simulink model "levitador_bola"  (R2023b)
settings: Solver=ode45  StartTime=0.0  StopTime=t_final  MaxStep=Ts/8  RelTol=1e-3
values from neighbouring files (symbols this model uses):
  folga = 45    [parametros_levitador.m]
  g = 9.81    [parametros_levitador.m]
  h_eq = [0     0.017 0.080 0.103 0.138 0.157 0.22 ]    [parametros_levitador.m]
  h_ini = 0.13    [parametros_levitador.m]
  K_v = 0.0063    [parametros_levitador.m]
  Kd = 250    [parametros_levitador.m]
  Ki = 5    [parametros_levitador.m]
  Kp = 130    [parametros_levitador.m]
  N_filtro = 25    [parametros_levitador.m]
  pwm_eq = [143.6 141.1 133.2 129.0 126.7 127.3 127.3]    [parametros_levitador.m]
  ruido_s = rd0    [analise_levitador.m]    (also in parametros_levitador.m = 6.25e-06)
  semente = 10*sem    [comparar_candidatos.m]    (also in parametros_levitador.m = 1)
  tau_v = 0.56    [parametros_levitador.m]
  Ts = 0.04    [parametros_levitador.m]
  turb_f = 0    [parametros_levitador.m]
  turb_sd = sd0    [analise_levitador.m]    (also in parametros_levitador.m = 4)
  u0 = 127    [parametros_levitador.m]
  u_max = 255    [parametros_levitador.m]
  u_min = 0    [parametros_levitador.m]
  v_ar_ini = K_v*pwm0    [parametros_levitador.m]
libraries: slpidlib x1
settings Model: Creator=autor  LastModifiedBy=autor

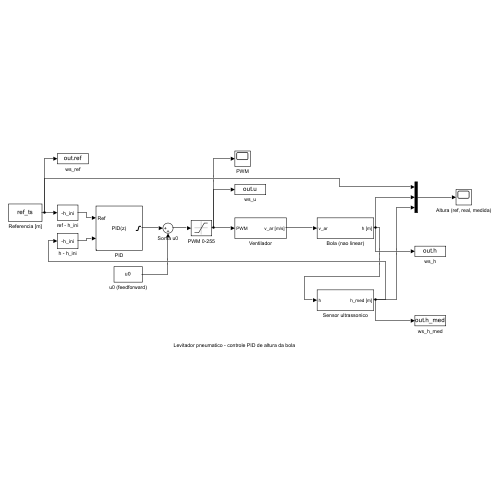
[thumbnail: Simulink's stored preview of the top-level diagram]
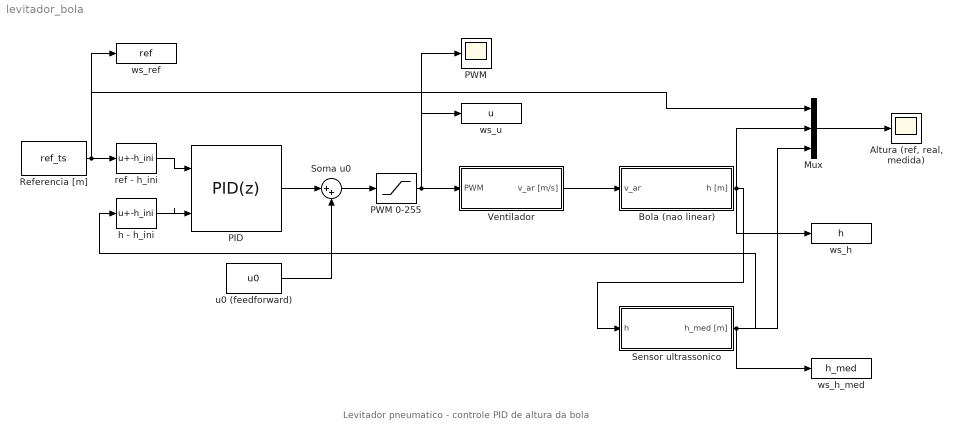
== system levitador_bola ==
  note: Levitador pneumatico - controle PID de altura da bola
  "Altura (ref, real, medida)" : Scope
  Bola (nao linear) : Subsystem
  Mux : Mux  Inputs=3
  PID : slpidlib/PID Controller (2DOF)  Controller=PID  Form=Parallel  TimeDomain=Discrete-time  UseExternalTs=off  SampleTime=Ts  IntegratorMethod=Forward Euler  FilterMethod=Backward Euler  ControllerParametersSource=internal  P=Kp  I=Ki  UseKiTs=off  D=Kd  N=N_filtro  UseFilter=on  b=1  c=0  TunerSelectOption=Transfer Function Based (PID Tuner App)  InitialConditionSource=internal  InitialConditionForIntegrator=0  InitialConditionForFilter=0  DifferentiatorICPrevScaledInput=0  ExternalReset=none  TrackingMode=off  Kt=1  LimitOutput=on  SatLimitsSource=internal  UpperSaturationLimit=folga  LowerSaturationLimit=u_min - u0  LinearizeAsGain=off  AntiWindupMode=clamping  Kb=1  LimitIntegrator=off  UpperIntegratorSaturationLimit=inf  LowerIntegratorSaturationLimit=-inf  POutMin=[]  POutMax=[]  IOutMin=[]  IOutMax=[]  DOutMin=[]  DOutMax=[]  NOutMin=[]  NOutMax=[]  bOutMin=[]  bOutMax=[]  cOutMin=[]  cOutMax=[]  SumOutMin=[]  SumOutMax=[]  SaturationOutMin=[]  SaturationOutMax=[]  PParamMin=[]  PParamMax=[]  IParamMin=[]  IParamMax=[]  DParamMin=[]  DParamMax=[]  NParamMin=[]  NParamMax=[]  bParamMin=[]  bParamMax=[]  cParamMin=[]  cParamMax=[]  KbParamMin=[]  KbParamMax=[]  KtParamMin=[]  KtParamMax=[]  KbOutMin=[]  KbOutMax=[]  KtOutMin=[]  KtOutMax=[]  IntegratorOutMin=[]  IntegratorOutMax=[]  FilterOutMin=[]  FilterOutMax=[]  SumI1OutMin=[]  SumI1OutMax=[]  SumI2OutMin=[]  SumI2OutMax=[]  SumI3OutMin=[]  SumI3OutMax=[]  SumI4OutMin=[]  SumI4OutMax=[]  SumDOutMin=[]  SumDOutMax=[]  Sum1OutMin=[]  Sum1OutMax=[]  Sum2OutMin=[]  Sum2OutMax=[]  Sum3OutMin=[]  Sum3OutMax=[]  DifferentiatorOutMin=[]  DifferentiatorOutMax=[]  FilterDiffOutCoefMin=[]  FilterDiffOutCoefMax=[]  ReciprocalOutMin=[]  ReciprocalOutMax=[]  SumDenOutMin=[]  SumDenOutMax=[]  SumNumOutMin=[]  SumNumOutMax=[]  DivideOutMin=[]  DivideOutMax=[]  UdiffTsProdOutMin=[]  UdiffTsProdOutMax=[]  NTsProdOutMin=[]  NTsProdOutMax=[]  UintegralTsProdOutMin=[]  UintegralTsProdOutMax=[]  UngainTsProdOutMin=[]  UngainTsProdOutMax=[]  ClampingZeroOutDataTypeStr=Inherit: Inherit via back propagation  ClampingZeroOutMin=[]  ClampingZeroOutMax=[]  FilterDenConstantOutDataTypeStr=Inherit: Inherit via back propagation  FilterDenConstantOutMin=[]  FilterDenConstantOutMax=[]  PCopyOutDataTypeStr=Inherit: Inherit via back propagation  PCopyOutMin=[]  PCopyOutMax=[]  NCopyOutDataTypeStr=Inherit: Inherit via back propagation  NCopyOutMin=[]  NCopyOutMax=[]  IntegratorContinuousStateAttributes=''  IntegratorStateMustResolveToSignalObject=off  IntegratorRTWStateStorageClass=Auto  FilterContinuousStateAttributes=''  FilterStateMustResolveToSignalObject=off  FilterRTWStateStorageClass=Auto  ParallelPVariant=InternalParameters  IdealPVariant=Disabled  IVariant=InternalParameters  DVariant=InternalParameters  bVariant=InternalParameters  cVariant=InternalParameters  IntegratorVariant=Discrete  SatVariant=Enabled  AWVariant=DiscClampingParallel  PCopyVariant=Disabled  TRVariant=Disabled  FdbkBlocksVariant=Forward  IdealPFdbkVariant=Disabled  SatFdbkVariant=Disabled  DerivativeFilterVariant=BackwardEulerFilter  NVariant=InternalParameters  NCopyVariant=InternalParameters  FilterICVariant=InternalICsFilter  IntegratorICVariant=InternalICs  ExternalResetVariant=Disabled  TRSumVariant=Passthrough  SumFdbkVariant=Disabled  SumVariant=Sum_PID  TsampFilterVariant=InternalTs  TsampNgainVariant=Passthrough  TsampIntegralVariant=Disabled_SignalSpec  ExternalSaturationOutDataTypeStr=Inherit: Same as second input
      settings: LibrarySourceBlock=simulink/Discrete/Discrete PID Controller (2DOF)
  PWM : Scope
  PWM 0-255 : Saturate  UpperLimit=u_max  LowerLimit=u_min
  Referencia [m] : FromWorkspace  VariableName=ref_ts  SampleTime=Ts  Interpolate=off  OutputAfterFinalValue=Holding final value
  Sensor ultrassonico : Subsystem
  Soma u0 : Sum  Inputs=|++
  Ventilador : Subsystem
  h - h_ini : Bias  Bias=-h_ini  SaturateOnIntegerOverflow=off
  ref - h_ini : Bias  Bias=-h_ini  SaturateOnIntegerOverflow=off
  u0 (feedforward) : Constant  Value=u0
  ws_h : ToWorkspace  VariableName=h  SaveFormat=Timeseries  SampleTime=Ts
  ws_h_med : ToWorkspace  VariableName=h_med  SaveFormat=Timeseries  SampleTime=Ts
  ws_ref : ToWorkspace  VariableName=ref  SaveFormat=Timeseries  SampleTime=Ts
  ws_u : ToWorkspace  VariableName=u  SaveFormat=Timeseries  SampleTime=Ts
  wires:
  Referencia [m]/1 -> ref - h_ini/1, Mux/1, ws_ref/1
  ref - h_ini/1 -> PID/1
  Sensor ultrassonico/1(h_med [m]) -> h - h_ini/1, Mux/3, ws_h_med/1
  h - h_ini/1 -> PID/2
  PID/1 -> Soma u0/1
  u0 (feedforward)/1 -> Soma u0/2
  Soma u0/1 -> PWM 0-255/1
  PWM 0-255/1 -> Ventilador/1(PWM), PWM/1, ws_u/1
  Ventilador/1(v_ar [m/s]) -> Bola (nao linear)/1(v_ar)
  Bola (nao linear)/1(h [m]) -> Sensor ultrassonico/1(h), Mux/2, ws_h/1
  Mux/1 -> "Altura (ref, real, medida)"/1

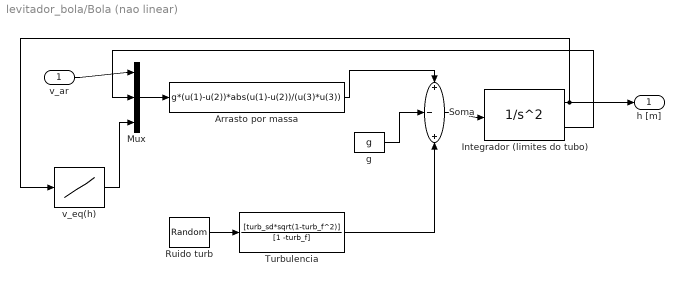
== system levitador_bola/Bola (nao linear) ==
  v_ar : Inport
  Arrasto por massa : Fcn  Expr=g*(u(1)-u(2))*abs(u(1)-u(2))/(u(3)*u(3))
  Integrador (limites do tubo) : SecondOrderIntegrator  ICX=h_ini  LimitX=on  UpperLimitX=h_max  LowerLimitX=0  ICDXDT=0  LimitDXDT=on
  Mux : Mux  Inputs=3
  Ruido turb : RandomNumber  Seed=semente  SampleTime=Ts
  Soma : Sum  Inputs=+-+
  Turbulencia : DiscreteTransferFcn  Numerator=[turb_sd*sqrt(1-turb_f^2)]  Denominator=[1 -turb_f]  SampleTime=Ts
  g : Constant  Value=g
  v_eq(h) : Lookup_n-D  NumberOfTableDimensions=1  BreakpointsForDimension1=h_eq  Table=K_v*pwm_eq  ExtrapMethod=Clip  InternalRulePriority=Speed  RndMeth=Simplest
  h [m] : Outport
  wires:
  v_ar/1 -> Mux/1
  v_eq(h)/1 -> Mux/3
  Mux/1 -> Arrasto por massa/1
  Arrasto por massa/1 -> Soma/1
  g/1 -> Soma/2
  Ruido turb/1 -> Turbulencia/1
  Turbulencia/1 -> Soma/3
  Soma/1 -> Integrador (limites do tubo)/1
  Integrador (limites do tubo)/1 -> h [m]/1, v_eq(h)/1
  Integrador (limites do tubo)/2 -> Mux/2

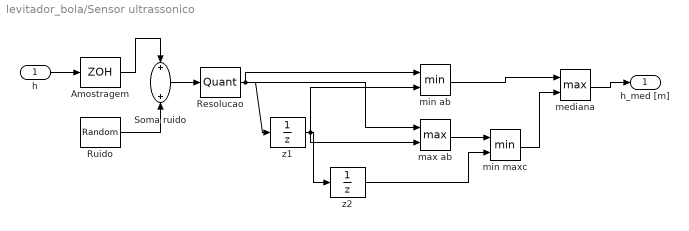
== system levitador_bola/Sensor ultrassonico ==
  h : Inport
  Amostragem : ZeroOrderHold  SampleTime=Ts
  Resolucao : Quantizer  QuantizationInterval=q_sens
  Ruido : RandomNumber  Variance=ruido_s  Seed=semente+1  SampleTime=Ts
  Soma ruido : Sum
  max ab : MinMax  Function=max  Inputs=2
  mediana : MinMax  Function=max  Inputs=2
  min ab : MinMax  Inputs=2
  min maxc : MinMax  Inputs=2
  z1 : UnitDelay  InitialCondition=h_ini  SampleTime=Ts  HasFrameUpgradeWarning=on
  z2 : UnitDelay  InitialCondition=h_ini  SampleTime=Ts  HasFrameUpgradeWarning=on
  h_med [m] : Outport
  wires:
  h/1 -> Amostragem/1
  Amostragem/1 -> Soma ruido/1
  Ruido/1 -> Soma ruido/2
  Soma ruido/1 -> Resolucao/1
  Resolucao/1 -> z1/1, min ab/1, max ab/1
  z1/1 -> z2/1, min ab/2, max ab/2
  max ab/1 -> min maxc/1
  z2/1 -> min maxc/2
  min ab/1 -> mediana/1
  min maxc/1 -> mediana/2
  mediana/1 -> h_med [m]/1

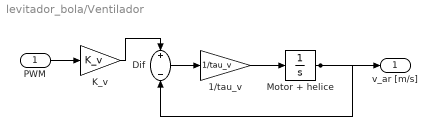
== system levitador_bola/Ventilador ==
  PWM : Inport
  1/tau_v : Gain  Gain=1/tau_v
  Dif : Sum  Inputs=+-
  K_v : Gain  Gain=K_v
  Motor + helice : Integrator  InitialCondition=v_ar_ini
  v_ar [m/s] : Outport
  wires:
  PWM/1 -> K_v/1
  K_v/1 -> Dif/1
  Dif/1 -> 1/tau_v/1
  1/tau_v/1 -> Motor + helice/1
  Motor + helice/1 -> v_ar [m/s]/1, Dif/2
